simulink model "afe_inv_psm_with_hf_models"  (R2026a)
settings: Solver=ode23tb  StopTime=simlength  FixedStep=tc  MaxStep=glb_time.tc
values from neighbouring files (symbols this model uses):
  afe_ctrl = ctrl_afe_setup(glb_time.ts_afe, grid_emu.omega_grid_nom)    [init_model.m]
  afe_pwm_phase_shift_mod1 = 0    [init_model.m]
  CTRPIFF_CLIP_RELEASE = 0.001    [init_model.m]
  DThs_init = 0    [init_model.m]
  filters = setup_global_filters(glb_time.ts_afe, glb_time.ts_inv, glb_time.ts_dab, glb_time.tc)    [init_model.m]
  frt_data = frt_settings(test_index, test_subindex, asymmetric_error_type,      enable_frt_1, enable_frt_2, start_time_LVRT, deepPOSxi, deepPOSeta, deepNEGxi, deepNEGeta)    [init_model.m]
  glb_time = timing_setup(fpwm_afe, trgo_afe, fpwm_inv, trgo_inv, fpwm_single_phase_inv, trgo_single_phase_inv, fpwm_dab, trgo_dab,      fpwm_psfbc, trgo_psfbc, fpwm_isop_rail, trgo_isop_rail, fpwm_cllc, trgo_cllc, t_measure, tc_factor, tc_decimation, delay_pwm, dead_time_afe,      dead_time_inv, dead_time_single_phase_inv, dead_time_dab, dead_time_psfbc, dead_time_isop_rail, dead_time_cllc)    [init_model.m]
  grid_emu = grid_three_phase_emulator('Dyn11', delta_star, grid_nominal_power, application_voltage, us1, us2, fgrid,                  eq_grid_inductance, eq_grid_resistance, eta, ucc, i1m, p_iron, n1, n2, core_area, core_length, mur,                  up_xi_pu_ref, up_eta_pu_ref, un_xi_pu_ref, un_eta_pu_ref)    [init_model.m]
  i_react_pos_ref_2 = -ixi_ref_mod1*tan(acos(0.95))    [init_model.m]
  i_react_pos_ref_3 = ixi_ref_mod1*tan(acos(0.95))    [init_model.m]
  inv_pwm_phase_shift_mod1 = 0    [init_model.m]
  ixi_ref_mod1 = -0.85    [init_model.m]
  ki_align = 18    [init_model.m]
  kp_align = 0.25    [init_model.m]
  lim_down_align = -0.05    [init_model.m]
  lim_up_align = 0.05    [init_model.m]
  mavarage_filter_frequency_base_order = 2    [init_model.m]
  omega_m_sim = psm.omega_m_bez    [init_model.m]
  psm = psm_calculus_with_variants(application_voltage)    [init_model.m]
  psm_ctrl = ctrl_pmsm_setup(glb_time.ts_inv, psm.omega_bez, u_psm_scale, psm.Jm_norm)    [init_model.m]
  rms_tc = rms_filter_setup(rms_tc_obj)    [init_model.m]
  simlength = 1.75    [init_model.m]
  Tambient = 40    [init_model.m]
  time_aux_power_supply_fault = 1e3    (= 1000)    [init_model.m]
  time_gain_afe_module_1 = 1.0002    [init_model.m]
  time_gain_inv_module_2 = 1.001    [init_model.m]
  time_i_react_pos_ref_1 = start_time_LVRT + error_length + 0.335    [init_model.m]
  time_i_react_pos_ref_2 = time_i_react_pos_ref_1 + 0.5    (= 0.5)    [init_model.m]
  time_start_motor_control = 0.25    [init_model.m]
  torque_overload_factor = 1    [init_model.m]
  u_cm_comp_mod1 = 0    [init_model.m]
  u_psm_scale_ekf = sqrt(3)/2 * 2/3 * hwdata.inv.udc_nom/psm.ubez    [init_model.m]
undefined symbols (not defined in the file or in its folder): hf_power_cable_model, hwdata, magnitude, omega_m_bez, rpm_base, torque_base
libraries: fl_lib x136, nesl_utility x57, moving_average_filter x10, moving_average_filter_cc x8, ee_lib x5, sl_discontinuities x3, single_phase_transformer_lib x3, linear_double_integrator_observer_ccaller x2, discrete_time_low_pass_filter x2, threephase_inductor_lib x2, three_phase_pwm_modulator x2, three_phase_inverter_ideal_switch_based_model x2
(part 4 of 10)

== system afe_inv_psm_with_hf_models/grid/grid_emulator/threephase_vi_measures ==
  Bus Creator : BusCreator  Inputs=6
  Current Sensor : fl_lib/Electrical/Electrical Sensors/Current Sensor
  Current Sensor1 : fl_lib/Electrical/Electrical Sensors/Current Sensor
  Current Sensor2 : fl_lib/Electrical/Electrical Sensors/Current Sensor
  Electrical Reference1 : fl_lib/Electrical/Electrical Elements/Electrical Reference
  Voltage Sensor : fl_lib/Electrical/Electrical Sensors/Voltage Sensor
  Voltage Sensor1 : fl_lib/Electrical/Electrical Sensors/Voltage Sensor
  Voltage Sensor2 : fl_lib/Electrical/Electrical Sensors/Voltage Sensor
  i : Selector  InputPortWidth=6  IndexOptions=Index vector (dialog)  Indices=[4 5 6]  OutputSizes=1
  ia_grid : nesl_utility/PS-Simulink Converter  PhysicalDomain=network_engine_domain  SubClassName=ps_output  LeftPortType=input  RightPortType=output  PseudoPeriodic=off  Frequencies=[]  VectorFormat=1-D array  Unit=A  AffineConversion=off
  ib_grid : nesl_utility/PS-Simulink Converter  PhysicalDomain=network_engine_domain  SubClassName=ps_output  LeftPortType=input  RightPortType=output  PseudoPeriodic=off  Frequencies=[]  VectorFormat=1-D array  Unit=A  AffineConversion=off
  ic_grid : nesl_utility/PS-Simulink Converter  PhysicalDomain=network_engine_domain  SubClassName=ps_output  LeftPortType=input  RightPortType=output  PseudoPeriodic=off  Frequencies=[]  VectorFormat=1-D array  Unit=A  AffineConversion=off
  u : Selector  InputPortWidth=6  IndexOptions=Index vector (dialog)  Indices=[1 2 3]  OutputSizes=1
  ua_grid : nesl_utility/PS-Simulink Converter  PhysicalDomain=network_engine_domain  SubClassName=ps_output  LeftPortType=input  RightPortType=output  PseudoPeriodic=off  Frequencies=[]  VectorFormat=1-D array  Unit=V  AffineConversion=off
  ub_grid : nesl_utility/PS-Simulink Converter  PhysicalDomain=network_engine_domain  SubClassName=ps_output  LeftPortType=input  RightPortType=output  PseudoPeriodic=off  Frequencies=[]  VectorFormat=1-D array  Unit=V  AffineConversion=off
  uc_grid : nesl_utility/PS-Simulink Converter  PhysicalDomain=network_engine_domain  SubClassName=ps_output  LeftPortType=input  RightPortType=output  PseudoPeriodic=off  Frequencies=[]  VectorFormat=1-D array  Unit=V  AffineConversion=off
  Ua : PMIOPort  Side=Left
  ua : PMIOPort  Port=2  Side=Right
  Ub : PMIOPort  Port=3  Side=Left
  ub : PMIOPort  Port=4  Side=Right
  Uc : PMIOPort  Port=5  Side=Left
  uc : PMIOPort  Port=6  Side=Right
  tag scope: i_abc_line=global, u_abc_line=global
  wires:
  Bus Creator/1 -> i/1, u/1  "vi_data"
  ib_grid/1 -> Bus Creator/5  "ib"
  ia_grid/1 -> Bus Creator/4  "ia"
  ic_grid/1 -> Bus Creator/6  "ic"
  ua_grid/1 -> Bus Creator/1  "ua"
  ub_grid/1 -> Bus Creator/2  "ub"
  uc_grid/1 -> Bus Creator/3  "uc"
  i/1 -> [i_abc_line]
  u/1 -> [u_abc_line]
  connections:
  Current Sensor1/LConn1 -- Ub/RConn1 -- Voltage Sensor1/LConn1
  Electrical Reference1/LConn1 -- Voltage Sensor/RConn2 -- Voltage Sensor2/RConn2 -- Voltage Sensor1/RConn2
  Voltage Sensor/RConn1 -- ua_grid/LConn1
  Current Sensor/RConn2 -- ua/RConn1
  Voltage Sensor1/RConn1 -- ub_grid/LConn1
  Voltage Sensor2/LConn1 -- Current Sensor2/LConn1 -- Uc/RConn1
  Current Sensor/LConn1 -- Ua/RConn1 -- Voltage Sensor/LConn1
  Current Sensor1/RConn2 -- ub/RConn1
  Voltage Sensor2/RConn1 -- uc_grid/LConn1
  ib_grid/LConn1 -- Current Sensor1/RConn1
  ia_grid/LConn1 -- Current Sensor/RConn1
  ic_grid/LConn1 -- Current Sensor2/RConn1
  Current Sensor2/RConn2 -- uc/RConn1

== system afe_inv_psm_with_hf_models/power_cables_and_psm_high_frequency_models/power_cable_model_1/parasitic_lump_1 ==
  Cp1 : fl_lib/Electrical/Electrical Elements/Capacitor  c=hf_power_cable_model.Cp1 F  r=hf_power_cable_model.RCs1 Ohm  g=0 1/Ohm  i_specify=off  i_priority=None  i=0 A  i_nominal_specify=off  i_nominal_value=1  i_nominal_unit=A  v_specify=off  v_priority=None  v=0 V  v_nominal_specify=off  v_nominal_value=1  v_nominal_unit=V  vc_specify=off  vc_priority=High  vc=0 V  vc_nominal_specify=off  vc_nominal_value=1  vc_nominal_unit=V
  Cp2 : fl_lib/Electrical/Electrical Elements/Capacitor  Commented=on  c=hf_power_cable_model.Cp2 F  r=hf_power_cable_model.RCs2 Ohm  g=0 1/Ohm  i_specify=off  i_priority=None  i=0 A  i_nominal_specify=off  i_nominal_value=1  i_nominal_unit=A  v_specify=off  v_priority=None  v=0 V  v_nominal_specify=off  v_nominal_value=1  v_nominal_unit=V  vc_specify=off  vc_priority=High  vc=0 V  vc_nominal_specify=off  vc_nominal_value=1  vc_nominal_unit=V
  Electrical Reference : fl_lib/Electrical/Electrical Elements/Electrical Reference
  Ls1 : fl_lib/Electrical/Electrical Elements/Inductor  l=hf_power_cable_model.Ls1 H  r=hf_power_cable_model.Rs1 Ohm  g=1e-9 1/Ohm  i_specify=off  i_priority=None  i=0 A  i_nominal_specify=off  i_nominal_value=1  i_nominal_unit=A  v_specify=off  v_priority=None  v=0 V  v_nominal_specify=off  v_nominal_value=1  v_nominal_unit=V  i_L_specify=off  i_L_priority=High  i_L=0 A  i_L_nominal_specify=off  i_L_nominal_value=1  i_L_nominal_unit=A
  Rp1 : fl_lib/Electrical/Electrical Elements/Resistor  Commented=on  R=hf_power_cable_model.Rp1 Ohm  i_specify=off  i_priority=None  i=0 A  i_nominal_specify=off  i_nominal_value=1  i_nominal_unit=A  v_specify=off  v_priority=None  v=0 V  v_nominal_specify=off  v_nominal_value=1  v_nominal_unit=V
  u1 : PMIOPort  Side=Left
  u2 : PMIOPort  Port=2  Side=Right
  connections:
  Ls1/LConn1 -- Cp2/LConn1 -- u1/RConn1
  Rp1/RConn1 -- Cp2/RConn1 -- Electrical Reference/LConn1 -- Cp1/RConn1
  u2/RConn1 -- Rp1/LConn1 -- Ls1/RConn1 -- Cp1/LConn1

== system afe_inv_psm_with_hf_models/power_cables_and_psm_high_frequency_models/power_cable_model_1/parasitic_lump_2 ==
  Cp1 : fl_lib/Electrical/Electrical Elements/Capacitor  c=hf_power_cable_model.Cp1 F  r=hf_power_cable_model.RCs1 Ohm  g=0 1/Ohm  i_specify=off  i_priority=None  i=0 A  i_nominal_specify=off  i_nominal_value=1  i_nominal_unit=A  v_specify=off  v_priority=None  v=0 V  v_nominal_specify=off  v_nominal_value=1  v_nominal_unit=V  vc_specify=off  vc_priority=High  vc=0 V  vc_nominal_specify=off  vc_nominal_value=1  vc_nominal_unit=V
  Cp2 : fl_lib/Electrical/Electrical Elements/Capacitor  Commented=on  c=hf_power_cable_model.Cp2 F  r=hf_power_cable_model.RCs2 Ohm  g=0 1/Ohm  i_specify=off  i_priority=None  i=0 A  i_nominal_specify=off  i_nominal_value=1  i_nominal_unit=A  v_specify=off  v_priority=None  v=0 V  v_nominal_specify=off  v_nominal_value=1  v_nominal_unit=V  vc_specify=off  vc_priority=High  vc=0 V  vc_nominal_specify=off  vc_nominal_value=1  vc_nominal_unit=V
  Electrical Reference : fl_lib/Electrical/Electrical Elements/Electrical Reference
  Ls1 : fl_lib/Electrical/Electrical Elements/Inductor  l=hf_power_cable_model.Ls1 H  r=hf_power_cable_model.Rs1 Ohm  g=1e-9 1/Ohm  i_specify=off  i_priority=None  i=0 A  i_nominal_specify=off  i_nominal_value=1  i_nominal_unit=A  v_specify=off  v_priority=None  v=0 V  v_nominal_specify=off  v_nominal_value=1  v_nominal_unit=V  i_L_specify=off  i_L_priority=High  i_L=0 A  i_L_nominal_specify=off  i_L_nominal_value=1  i_L_nominal_unit=A
  Rp1 : fl_lib/Electrical/Electrical Elements/Resistor  Commented=on  R=hf_power_cable_model.Rp1 Ohm  i_specify=off  i_priority=None  i=0 A  i_nominal_specify=off  i_nominal_value=1  i_nominal_unit=A  v_specify=off  v_priority=None  v=0 V  v_nominal_specify=off  v_nominal_value=1  v_nominal_unit=V
  u1 : PMIOPort  Side=Left
  u2 : PMIOPort  Port=2  Side=Right
  connections:
  Cp1/LConn1 -- Ls1/RConn1 -- Rp1/LConn1 -- u2/RConn1
  Cp1/RConn1 -- Electrical Reference/LConn1 -- Cp2/RConn1 -- Rp1/RConn1
  u1/RConn1 -- Cp2/LConn1 -- Ls1/LConn1

== system afe_inv_psm_with_hf_models/power_cables_and_psm_high_frequency_models/power_cable_model_2/parasitic_lump_1 ==
  Cp1 : fl_lib/Electrical/Electrical Elements/Capacitor  c=hf_power_cable_model.Cp1 F  r=hf_power_cable_model.RCs1 Ohm  g=0 1/Ohm  i_specify=off  i_priority=None  i=0 A  i_nominal_specify=off  i_nominal_value=1  i_nominal_unit=A  v_specify=off  v_priority=None  v=0 V  v_nominal_specify=off  v_nominal_value=1  v_nominal_unit=V  vc_specify=off  vc_priority=High  vc=0 V  vc_nominal_specify=off  vc_nominal_value=1  vc_nominal_unit=V
  Cp2 : fl_lib/Electrical/Electrical Elements/Capacitor  Commented=on  c=hf_power_cable_model.Cp2 F  r=hf_power_cable_model.RCs2 Ohm  g=0 1/Ohm  i_specify=off  i_priority=None  i=0 A  i_nominal_specify=off  i_nominal_value=1  i_nominal_unit=A  v_specify=off  v_priority=None  v=0 V  v_nominal_specify=off  v_nominal_value=1  v_nominal_unit=V  vc_specify=off  vc_priority=High  vc=0 V  vc_nominal_specify=off  vc_nominal_value=1  vc_nominal_unit=V
  Electrical Reference : fl_lib/Electrical/Electrical Elements/Electrical Reference
  Ls1 : fl_lib/Electrical/Electrical Elements/Inductor  l=hf_power_cable_model.Ls1 H  r=hf_power_cable_model.Rs1 Ohm  g=1e-9 1/Ohm  i_specify=off  i_priority=None  i=0 A  i_nominal_specify=off  i_nominal_value=1  i_nominal_unit=A  v_specify=off  v_priority=None  v=0 V  v_nominal_specify=off  v_nominal_value=1  v_nominal_unit=V  i_L_specify=off  i_L_priority=High  i_L=0 A  i_L_nominal_specify=off  i_L_nominal_value=1  i_L_nominal_unit=A
  Rp1 : fl_lib/Electrical/Electrical Elements/Resistor  Commented=on  R=hf_power_cable_model.Rp1 Ohm  i_specify=off  i_priority=None  i=0 A  i_nominal_specify=off  i_nominal_value=1  i_nominal_unit=A  v_specify=off  v_priority=None  v=0 V  v_nominal_specify=off  v_nominal_value=1  v_nominal_unit=V
  u1 : PMIOPort  Side=Left
  u2 : PMIOPort  Port=2  Side=Right
  connections:
  Cp1/LConn1 -- Ls1/RConn1 -- Rp1/LConn1 -- u2/RConn1
  Cp1/RConn1 -- Electrical Reference/LConn1 -- Cp2/RConn1 -- Rp1/RConn1
  u1/RConn1 -- Cp2/LConn1 -- Ls1/LConn1

== system afe_inv_psm_with_hf_models/power_cables_and_psm_high_frequency_models/power_cable_model_2/parasitic_lump_2 ==
  Cp1 : fl_lib/Electrical/Electrical Elements/Capacitor  c=hf_power_cable_model.Cp1 F  r=hf_power_cable_model.RCs1 Ohm  g=0 1/Ohm  i_specify=off  i_priority=None  i=0 A  i_nominal_specify=off  i_nominal_value=1  i_nominal_unit=A  v_specify=off  v_priority=None  v=0 V  v_nominal_specify=off  v_nominal_value=1  v_nominal_unit=V  vc_specify=off  vc_priority=High  vc=0 V  vc_nominal_specify=off  vc_nominal_value=1  vc_nominal_unit=V
  Cp2 : fl_lib/Electrical/Electrical Elements/Capacitor  Commented=on  c=hf_power_cable_model.Cp2 F  r=hf_power_cable_model.RCs2 Ohm  g=0 1/Ohm  i_specify=off  i_priority=None  i=0 A  i_nominal_specify=off  i_nominal_value=1  i_nominal_unit=A  v_specify=off  v_priority=None  v=0 V  v_nominal_specify=off  v_nominal_value=1  v_nominal_unit=V  vc_specify=off  vc_priority=High  vc=0 V  vc_nominal_specify=off  vc_nominal_value=1  vc_nominal_unit=V
  Electrical Reference : fl_lib/Electrical/Electrical Elements/Electrical Reference
  Ls1 : fl_lib/Electrical/Electrical Elements/Inductor  l=hf_power_cable_model.Ls1 H  r=hf_power_cable_model.Rs1 Ohm  g=1e-9 1/Ohm  i_specify=off  i_priority=None  i=0 A  i_nominal_specify=off  i_nominal_value=1  i_nominal_unit=A  v_specify=off  v_priority=None  v=0 V  v_nominal_specify=off  v_nominal_value=1  v_nominal_unit=V  i_L_specify=off  i_L_priority=High  i_L=0 A  i_L_nominal_specify=off  i_L_nominal_value=1  i_L_nominal_unit=A
  Rp1 : fl_lib/Electrical/Electrical Elements/Resistor  Commented=on  R=hf_power_cable_model.Rp1 Ohm  i_specify=off  i_priority=None  i=0 A  i_nominal_specify=off  i_nominal_value=1  i_nominal_unit=A  v_specify=off  v_priority=None  v=0 V  v_nominal_specify=off  v_nominal_value=1  v_nominal_unit=V
  u1 : PMIOPort  Side=Left
  u2 : PMIOPort  Port=2  Side=Right
  connections:
  Ls1/LConn1 -- Cp2/LConn1 -- u1/RConn1
  Cp2/RConn1 -- Electrical Reference/LConn1 -- Rp1/RConn1 -- Cp1/RConn1
  u2/RConn1 -- Rp1/LConn1 -- Ls1/RConn1 -- Cp1/LConn1

== system afe_inv_psm_with_hf_models/power_cables_and_psm_high_frequency_models/power_cable_model_3/parasitic_lump_1 ==
  Cp1 : fl_lib/Electrical/Electrical Elements/Capacitor  c=hf_power_cable_model.Cp1 F  r=hf_power_cable_model.RCs1 Ohm  g=0 1/Ohm  i_specify=off  i_priority=None  i=0 A  i_nominal_specify=off  i_nominal_value=1  i_nominal_unit=A  v_specify=off  v_priority=None  v=0 V  v_nominal_specify=off  v_nominal_value=1  v_nominal_unit=V  vc_specify=off  vc_priority=High  vc=0 V  vc_nominal_specify=off  vc_nominal_value=1  vc_nominal_unit=V
  Cp2 : fl_lib/Electrical/Electrical Elements/Capacitor  Commented=on  c=hf_power_cable_model.Cp2 F  r=hf_power_cable_model.RCs2 Ohm  g=0 1/Ohm  i_specify=off  i_priority=None  i=0 A  i_nominal_specify=off  i_nominal_value=1  i_nominal_unit=A  v_specify=off  v_priority=None  v=0 V  v_nominal_specify=off  v_nominal_value=1  v_nominal_unit=V  vc_specify=off  vc_priority=High  vc=0 V  vc_nominal_specify=off  vc_nominal_value=1  vc_nominal_unit=V
  Electrical Reference : fl_lib/Electrical/Electrical Elements/Electrical Reference
  Ls1 : fl_lib/Electrical/Electrical Elements/Inductor  l=hf_power_cable_model.Ls1 H  r=hf_power_cable_model.Rs1 Ohm  g=1e-9 1/Ohm  i_specify=off  i_priority=None  i=0 A  i_nominal_specify=off  i_nominal_value=1  i_nominal_unit=A  v_specify=off  v_priority=None  v=0 V  v_nominal_specify=off  v_nominal_value=1  v_nominal_unit=V  i_L_specify=off  i_L_priority=High  i_L=0 A  i_L_nominal_specify=off  i_L_nominal_value=1  i_L_nominal_unit=A
  Rp1 : fl_lib/Electrical/Electrical Elements/Resistor  Commented=on  R=hf_power_cable_model.Rp1 Ohm  i_specify=off  i_priority=None  i=0 A  i_nominal_specify=off  i_nominal_value=1  i_nominal_unit=A  v_specify=off  v_priority=None  v=0 V  v_nominal_specify=off  v_nominal_value=1  v_nominal_unit=V
  u1 : PMIOPort  Side=Left
  u2 : PMIOPort  Port=2  Side=Right
  connections:
  Ls1/LConn1 -- Cp2/LConn1 -- u1/RConn1
  Cp2/RConn1 -- Electrical Reference/LConn1 -- Rp1/RConn1 -- Cp1/RConn1
  u2/RConn1 -- Rp1/LConn1 -- Ls1/RConn1 -- Cp1/LConn1

== system afe_inv_psm_with_hf_models/power_cables_and_psm_high_frequency_models/power_cable_model_3/parasitic_lump_2 ==
  Cp1 : fl_lib/Electrical/Electrical Elements/Capacitor  c=hf_power_cable_model.Cp1 F  r=hf_power_cable_model.RCs1 Ohm  g=0 1/Ohm  i_specify=off  i_priority=None  i=0 A  i_nominal_specify=off  i_nominal_value=1  i_nominal_unit=A  v_specify=off  v_priority=None  v=0 V  v_nominal_specify=off  v_nominal_value=1  v_nominal_unit=V  vc_specify=off  vc_priority=High  vc=0 V  vc_nominal_specify=off  vc_nominal_value=1  vc_nominal_unit=V
  Cp2 : fl_lib/Electrical/Electrical Elements/Capacitor  Commented=on  c=hf_power_cable_model.Cp2 F  r=hf_power_cable_model.RCs2 Ohm  g=0 1/Ohm  i_specify=off  i_priority=None  i=0 A  i_nominal_specify=off  i_nominal_value=1  i_nominal_unit=A  v_specify=off  v_priority=None  v=0 V  v_nominal_specify=off  v_nominal_value=1  v_nominal_unit=V  vc_specify=off  vc_priority=High  vc=0 V  vc_nominal_specify=off  vc_nominal_value=1  vc_nominal_unit=V
  Electrical Reference : fl_lib/Electrical/Electrical Elements/Electrical Reference
  Ls1 : fl_lib/Electrical/Electrical Elements/Inductor  l=hf_power_cable_model.Ls1 H  r=hf_power_cable_model.Rs1 Ohm  g=1e-9 1/Ohm  i_specify=off  i_priority=None  i=0 A  i_nominal_specify=off  i_nominal_value=1  i_nominal_unit=A  v_specify=off  v_priority=None  v=0 V  v_nominal_specify=off  v_nominal_value=1  v_nominal_unit=V  i_L_specify=off  i_L_priority=High  i_L=0 A  i_L_nominal_specify=off  i_L_nominal_value=1  i_L_nominal_unit=A
  Rp1 : fl_lib/Electrical/Electrical Elements/Resistor  Commented=on  R=hf_power_cable_model.Rp1 Ohm  i_specify=off  i_priority=None  i=0 A  i_nominal_specify=off  i_nominal_value=1  i_nominal_unit=A  v_specify=off  v_priority=None  v=0 V  v_nominal_specify=off  v_nominal_value=1  v_nominal_unit=V
  u1 : PMIOPort  Side=Left
  u2 : PMIOPort  Port=2  Side=Right
  connections:
  Cp1/LConn1 -- Ls1/RConn1 -- Rp1/LConn1 -- u2/RConn1
  Cp1/RConn1 -- Rp1/RConn1 -- Electrical Reference/LConn1 -- Cp2/RConn1
  u1/RConn1 -- Cp2/LConn1 -- Ls1/LConn1

== system afe_inv_psm_with_hf_models/scopes/cable_effects/rms ==
  in : Inport
  Gain : Gain  Gain=rms_tc.n1-1
  Gain1 : Gain  Gain=1/rms_tc.n1
  Math Function : Math  Operator=magnitude^2  SignedPower=on
  Sqrt : Sqrt
  Sum : Sum  Inputs=|++
  Unit Delay : UnitDelay  SampleTime=glb_time.tc
  out : Outport  VectorParamsAs1DForOutWhenUnconnected=off
  wires:
  in/1 -> Math Function/1
  Sum/1 -> Gain1/1
  Gain1/1 -> Sqrt/1, Unit Delay/1
  Unit Delay/1 -> Gain/1
  Math Function/1 -> Sum/1
  Sqrt/1 -> out/1
  Gain/1 -> Sum/2

== system afe_inv_psm_with_hf_models/afe_abc_inv_psm_mod1/AFE_control/afe_control/FRT-VDE4110 ==
  Constant : Constant  Value=0
  FRT-Detection : Subsystem
  FRT-PosNegReactiveCurrentReferences : Subsystem
  Terminator : Terminator
  Terminator1 : Terminator
  frt_detection_output : Scope  NumInputPorts=3
      settings: ActiveDisplayYMinimum=-0.12499999999999997  ActiveDisplayYMaximum=1.125
  tag scope: frt_active=scoped, pwr_lim_enable=scoped
  wires:
  [v_grid_pos_xi_avg] -> FRT-PosNegReactiveCurrentReferences/1(In1)
  [v_grid_neg_xi_avg] -> FRT-PosNegReactiveCurrentReferences/3(In3)
  [v_grid_neg_eta_avg] -> FRT-PosNegReactiveCurrentReferences/4(In4)
  [v_grid_pos_eta_avg] -> FRT-PosNegReactiveCurrentReferences/2(In2)
  FRT-Detection/4(frt_active) -> frt_detection_output/2, [frt_active]  "frt_active"
  FRT-Detection/5(pwr_lim_enable) -> frt_detection_output/3, [pwr_lim_enable]  "pwr_lim_enable"
  FRT-Detection/2(frt_state) -> frt_detection_output/1  "frt_state"
  Constant/1 -> FRT-Detection/1(red_dyn_enabled)
  FRT-Detection/1(frt_exceeded) -> Terminator/1
  FRT-Detection/3(red_dyn_active) -> Terminator1/1

== system afe_inv_psm_with_hf_models/afe_abc_inv_psm_mod1/AFE_control/afe_control/current_ctrl ==
  i_xi_ref : Inport
  Demux : Demux  Outputs=3
  current_transformation : Subsystem
  inner_current_ctrl : Subsystem
  xieta2abc : Subsystem
  uabg_out : Outport
  wires:
  Demux/1 -> current_transformation/1(is_a_pu)  "is_a"
  Demux/2 -> current_transformation/2(is_b_pu)  "is_b"
  Demux/3 -> current_transformation/3(is_c_pu)  "is_c"
  [isd_abc_pu] -> Demux/1
  [phase_grid_pll] -> xieta2abc/5(phase)
  xieta2abc/1(i_abc) -> inner_current_ctrl/1(In1)
  [isd_abc_pu] -> inner_current_ctrl/2(is_abc)
  inner_current_ctrl/1(uabg) -> uabg_out/1
  i_xi_ref/1 -> xieta2abc/1(pos_xi)  "i_xi_ref"
  [i_stack_neg_eta_ref] -> xieta2abc/4(neg_eta)
  [i_stack_neg_xi_ref] -> xieta2abc/3(neg_xi)
  [i_stack_pos_eta_ref] -> xieta2abc/2(pos_eta)

== system afe_inv_psm_with_hf_models/afe_abc_inv_psm_mod1/AFE_control/afe_control/data_to_worspace_module_1 ==
  Bus Creator : BusCreator  Inputs=5
  dq_pll : Subsystem
  inner_current_tracking : Subsystem
  pwr_meter : Subsystem
  sequences_data : Subsystem
  m : Outport
  wires:
  Bus Creator/1 -> m/1
  sequences_data/1(m_seq) -> Bus Creator/1  "sequences_data"
  pwr_meter/1(m_pwr_meter) -> Bus Creator/2  "pwr_meter"
  inner_current_tracking/1(m_inner_current_tracking) -> Bus Creator/3  "m_inner_current_tracking"
  [local_time] -> Bus Creator/5  "local_time"
  dq_pll/1(dqPLLs) -> Bus Creator/4  "dq_pll"

== system afe_inv_psm_with_hf_models/afe_abc_inv_psm_mod1/AFE_control/afe_control/grid_current_sequences_and_reactive_pwr_ctrl ==
  ig_abc_pu : Inport
  current_sequence_avg : Subsystem
  grid_current_sampling_and_alpha_beta_transformation : Subsystem
  i_alphabeta2xieta : Subsystem
  sequences_current_control : Subsystem
  tag scope: i_grid_neg_eta_avg=scoped, i_grid_neg_xi_avg=scoped, i_grid_pos_eta_avg=scoped, i_grid_pos_xi_avg=scoped
  wires:
  i_alphabeta2xieta/1(xi) -> current_sequence_avg/1(i_grid_pos_xi)
  i_alphabeta2xieta/3(v_grid_neg_xi) -> current_sequence_avg/3(i_grid_neg_xi)
  i_alphabeta2xieta/4(e) -> current_sequence_avg/4(i_grid_neg_eta)
  current_sequence_avg/4(i_grid_neg_eta_avg) -> sequences_current_control/4(i_neg_eta), [i_grid_neg_eta_avg]
  ig_abc_pu/1 -> grid_current_sampling_and_alpha_beta_transformation/1(ig_abc)
  i_alphabeta2xieta/2(v_grid_pos_eta) -> current_sequence_avg/2(i_grid_pos_eta)
  current_sequence_avg/1(i_grid_pos_xi_avg) -> [i_grid_pos_xi_avg], sequences_current_control/1(i_pos_xi)
  current_sequence_avg/2(i_grid_pos_eta_avg) -> [i_grid_pos_eta_avg], sequences_current_control/2(i_pos_eta)
  [phase_grid_pll] -> i_alphabeta2xieta/3(gamma)
  grid_current_sampling_and_alpha_beta_transformation/2(i_grid_beta) -> i_alphabeta2xieta/2(beta)
  grid_current_sampling_and_alpha_beta_transformation/1(i_grid_alpha) -> i_alphabeta2xieta/1(alpha)
  current_sequence_avg/3(i_grid_neg_xi_avg) -> sequences_current_control/3(i_neg_xi), [i_grid_neg_xi_avg]

== system afe_inv_psm_with_hf_models/afe_abc_inv_psm_mod1/AFE_control/afe_control/grid_phase_acquisition ==
  grid_phase : Inport
  Quantizer : Quantizer  QuantizationInterval=adc_quantization
  Unit Delay : UnitDelay  SampleTime=-1
  Zero-Order Hold : ZeroOrderHold  SampleTime=-1
  grid_phased : Outport
  wires:
  Zero-Order Hold/1 -> Quantizer/1
  Unit Delay/1 -> grid_phased/1
  grid_phase/1 -> Zero-Order Hold/1
  Quantizer/1 -> Unit Delay/1

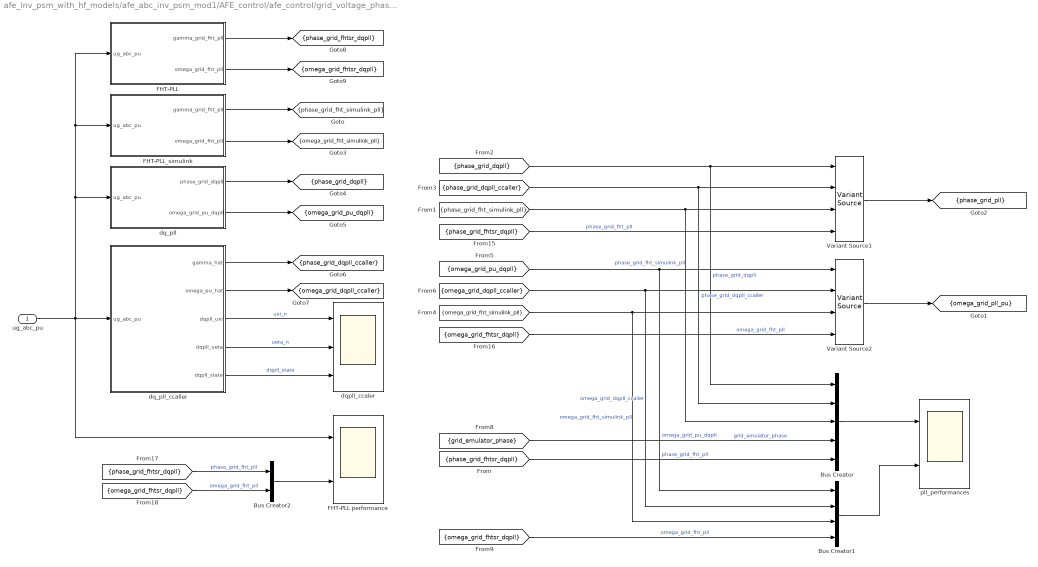
== system afe_inv_psm_with_hf_models/afe_abc_inv_psm_mod1/AFE_control/afe_control/grid_voltage_phase_lock_loops ==
  ug_abc_pu : Inport
  Bus Creator : BusCreator  Inputs=5
  Bus Creator1 : BusCreator  Inputs=4
  Bus Creator2 : BusCreator  Inputs=2
  FHT-PLL : Subsystem
  FHT-PLL performance : Scope  NumInputPorts=2
      settings: ActiveDisplayYMinimum=-1.251220703125  ActiveDisplayYMaximum=1.251220703125  DataLoggingVariableName=ScopeData8
  FHT-PLL_simulink : Subsystem
  Variant Source1 : VariantSource  VariantControls={use_dq_pll_mode1 == 1, use_dq_pll_mode2 == 1, use_dq_pll_mode3 == 1, use_dq_pll_mode4 == 1}
  Variant Source2 : VariantSource  VariantControls={use_dq_pll_mode1 == 1, use_dq_pll_mode2 == 1, use_dq_pll_mode3 == 1, use_dq_pll_mode4 == 1}
  dq_pll : Subsystem
  dq_pll_ccaller : Subsystem
  dqpll_ccaler : Scope  NumInputPorts=3
      settings: ActiveDisplayYMinimum=-0.88802937790751446  ActiveDisplayYMaximum=4.5431143753230572  DataLoggingVariableName=ScopeData4
  pll_performances : Scope  NumInputPorts=2
      settings: ActiveDisplayYMinimum=-3.9264641704366507  ActiveDisplayYMaximum=3.9264746341683896  DataLoggingVariableName=ScopeData34
  tag scope: omega_grid_dqpll_ccaller=scoped, omega_grid_fht_simulink_pll=scoped, omega_grid_fhtsr_dqpll=scoped, omega_grid_pll_pu=scoped, omega_grid_pu_dqpll=scoped, phase_grid_dqpll=scoped, phase_grid_dqpll_ccaller=scoped, phase_grid_fht_simulink_pll=scoped, phase_grid_fhtsr_dqpll=scoped, phase_grid_pll=scoped
  wires:
  Variant Source1/1 -> [phase_grid_pll]
  FHT-PLL_simulink/1(gamma_grid_fht_pll) -> [phase_grid_fht_simulink_pll]
  FHT-PLL_simulink/2(omega_grid_fht_pll) -> [omega_grid_fht_simulink_pll]
  dq_pll/2(omega_grid_pu_dqpll) -> [omega_grid_pu_dqpll]
  dq_pll/1(phase_grid_dqpll) -> [phase_grid_dqpll]
  dq_pll_ccaller/1(gamma_hat) -> [phase_grid_dqpll_ccaller]
  dq_pll_ccaller/2(omega_pu_hat) -> [omega_grid_dqpll_ccaller]
  [phase_grid_dqpll] -> Variant Source1/1, Bus Creator/1  "phase_grid_dqpll"
  [phase_grid_dqpll_ccaller] -> Bus Creator/2, Variant Source1/2  "phase_grid_dqpll_ccaller"
  [phase_grid_fht_simulink_pll] -> Bus Creator/3, Variant Source1/3  "phase_grid_fht_simulink_pll"
  [omega_grid_pu_dqpll] -> Variant Source2/1, Bus Creator1/1  "omega_grid_pu_dqpll"
  [omega_grid_dqpll_ccaller] -> Variant Source2/2, Bus Creator1/2  "omega_grid_dqpll_ccaller"
  [omega_grid_fht_simulink_pll] -> Variant Source2/3, Bus Creator1/3  "omega_grid_fht_simulink_pll"
  Variant Source2/1 -> [omega_grid_pll_pu]
  dq_pll_ccaller/3(dqpll_uxi) -> dqpll_ccaler/1  "uxi_n"
  dq_pll_ccaller/4(dqpll_ueta) -> dqpll_ccaler/2  "ueta_n"
  dq_pll_ccaller/5(dqpll_state) -> dqpll_ccaler/3  "dqpll_state"
  ug_abc_pu/1 -> FHT-PLL performance/1, dq_pll/1(ug_abc_pu), FHT-PLL_simulink/1(ug_abc_pu), FHT-PLL/1(ug_abc_pu), dq_pll_ccaller/1(ug_abc_pu)
  Bus Creator/1 -> pll_performances/1
  Bus Creator1/1 -> pll_performances/2
  [grid_emulator_phase] -> Bus Creator/4  "grid_emulator_phase"
  FHT-PLL/2(omega_grid_fht_pll) -> [omega_grid_fhtsr_dqpll]
  FHT-PLL/1(gamma_grid_fht_pll) -> [phase_grid_fhtsr_dqpll]
  [phase_grid_fhtsr_dqpll] -> Bus Creator/5  "phase_grid_fht_pll"
  [omega_grid_fhtsr_dqpll] -> Bus Creator1/4  "omega_grid_fht_pll"
  [phase_grid_fhtsr_dqpll] -> Variant Source1/4  "phase_grid_fht_pll"
  [omega_grid_fhtsr_dqpll] -> Variant Source2/4  "omega_grid_fht_pll"
  Bus Creator2/1 -> FHT-PLL performance/2
  [omega_grid_fhtsr_dqpll] -> Bus Creator2/2  "omega_grid_fht_pll"
  [phase_grid_fhtsr_dqpll] -> Bus Creator2/1  "phase_grid_fht_pll"

== system afe_inv_psm_with_hf_models/afe_abc_inv_psm_mod1/AFE_control/afe_control/grid_voltage_sequences ==
  grid_voltage_sampling_and_alpha_beta_transformation : Subsystem
  v_alphabeta2xieta : Subsystem
  voltage_sequence_avg : Subsystem
  tag scope: ug_alpha_pu=scoped, ug_beta_pu=scoped, v_grid_neg_eta_avg=scoped, v_grid_neg_xi_avg=scoped, v_grid_pos_eta_avg=scoped, v_grid_pos_xi_avg=scoped
  wires:
  v_alphabeta2xieta/4(v_grid_neg_eta) -> voltage_sequence_avg/4(v_grid_neg_eta)  "neg_eta"
  v_alphabeta2xieta/2(eta) -> voltage_sequence_avg/2(v_grid_pos_eta)  "pos_eta"
  [phase_grid_pll] -> v_alphabeta2xieta/3(gamma)
  v_alphabeta2xieta/3(v_grid_neg_xi) -> voltage_sequence_avg/3(v_grid_neg_xi)  "neg_xi"
  voltage_sequence_avg/3(v_grid_neg_xi_avg) -> [v_grid_neg_xi_avg]
  voltage_sequence_avg/2(v_grid_pos_eta_avg) -> [v_grid_pos_eta_avg]
  voltage_sequence_avg/4(v_grid_neg_eta_avg) -> [v_grid_neg_eta_avg]
  grid_voltage_sampling_and_alpha_beta_transformation/2(u_grid_beta) -> [ug_beta_pu], v_alphabeta2xieta/2(beta)
  voltage_sequence_avg/1(v_grid_pos_xi_avg) -> [v_grid_pos_xi_avg]
  v_alphabeta2xieta/1(xi) -> voltage_sequence_avg/1(v_grid_pos_xi)  "pos_xi"
  grid_voltage_sampling_and_alpha_beta_transformation/1(u_grid_alpha) -> [ug_alpha_pu], v_alphabeta2xieta/1(alpha)
  [ugd_abc_pu] -> grid_voltage_sampling_and_alpha_beta_transformation/1(v_abc)

== system afe_inv_psm_with_hf_models/afe_abc_inv_psm_mod1/AFE_control/afe_control/i_xi_ref ==
  Constant1 : Constant  Value=ixi_ref_mod1
  Constant2 : Constant  Value=0
  Delay : Delay  DelayLength=floor(0.25/glb_time.ts_afe)
  Switch : Switch  Criteria=u2 > Threshold  SaturateOnIntegerOverflow=off  InputSameDT=off
  Switch1 : Switch  Criteria=u2 > Threshold  SaturateOnIntegerOverflow=off  InputSameDT=off
  Variant Source : VariantSource  VariantControls={false, true}
  discrete-time-low-pass-filter : discrete_time_low_pass_filter/discrete-time-low-pass-filter  tau=0.125  ts=glb_time.ts_afe
  i_xi_ref : Outport
  wires:
  Constant1/1 -> Switch/3  "i_xi_ref"
  Constant2/1 -> Switch/1
  [pwr_lim_enable] -> Switch/2
  [pwr_lim_enable] -> Delay/1
  Switch/1 -> discrete-time-low-pass-filter/1, Variant Source/2, Switch1/3
  Delay/1 -> Switch1/2
  discrete-time-low-pass-filter/1 -> Switch1/1
  Switch1/1 -> Variant Source/1
  Variant Source/1 -> i_xi_ref/1

== system afe_inv_psm_with_hf_models/afe_abc_inv_psm_mod1/AFE_control/afe_control/ig afe quantizzation and one step delay ==
  ig_abc_pu : Inport
  Demux1 : Demux  Outputs=3
  Mux1 : Mux  Inputs=3
  ig afe quantizzation and one step delay : Subsystem
  igd_abc_pu : Outport
  wires:
  Demux1/1 -> ig afe quantizzation and one step delay/1(ig_u_pu)
  Demux1/2 -> ig afe quantizzation and one step delay/2(ig_v_pu)
  ig_abc_pu/1 -> Demux1/1
  Mux1/1 -> igd_abc_pu/1
  Demux1/3 -> ig afe quantizzation and one step delay/3(ig_w_pu)
  ig afe quantizzation and one step delay/2(igd_v_pu) -> Mux1/2
  ig afe quantizzation and one step delay/1(igd_u_pu) -> Mux1/1
  ig afe quantizzation and one step delay/3(igd_w_pu) -> Mux1/3

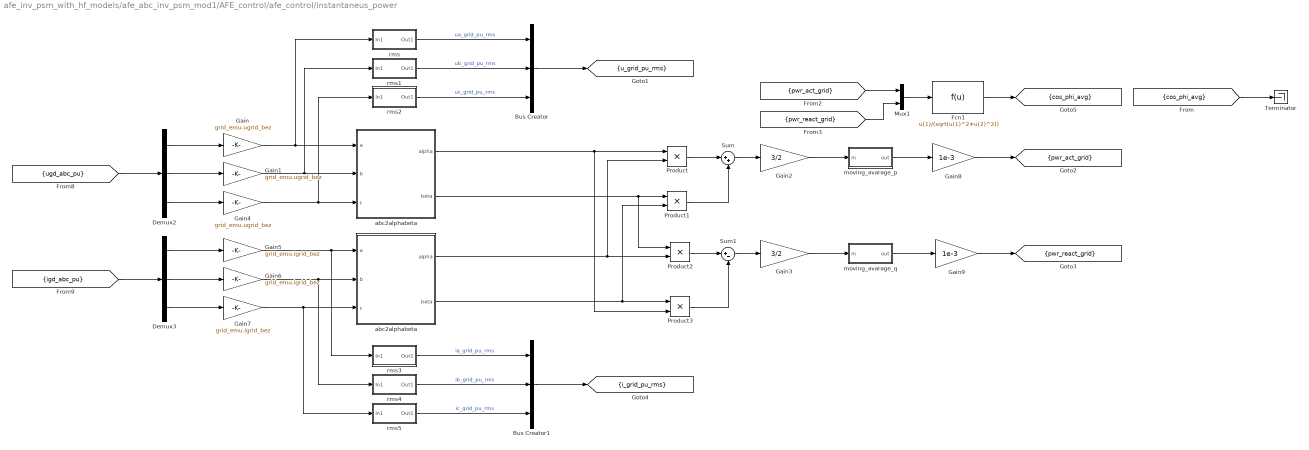
== system afe_inv_psm_with_hf_models/afe_abc_inv_psm_mod1/AFE_control/afe_control/instantaneus_power ==
  Bus Creator : BusCreator  Inputs=3
  Bus Creator1 : BusCreator  Inputs=3
  Demux2 : Demux  Outputs=3
  Demux3 : Demux  Outputs=3
  Fcn1 : Fcn  Expr=u(1)/(sqrt(u(1)^2+u(2)^2))
  Gain : Gain  Gain=grid_emu.ugrid_bez
  Gain1 : Gain  Gain=grid_emu.ugrid_bez
  Gain2 : Gain  Gain=3/2
  Gain3 : Gain  Gain=3/2
  Gain4 : Gain  Gain=grid_emu.ugrid_bez
  Gain5 : Gain  Gain=grid_emu.igrid_bez
  Gain6 : Gain  Gain=grid_emu.igrid_bez
  Gain7 : Gain  Gain=grid_emu.igrid_bez
  Gain8 : Gain  Gain=1e-3
  Gain9 : Gain  Gain=1e-3
  Mux1 : Mux  Inputs=2
  Product{,1..3} (4 alike) : Product  RndMeth=Zero
  Sum : Sum  Inputs=|++
  Sum1 : Sum  Inputs=|+-
  Terminator : Terminator
  abc2alphabeta : Subsystem
  "abc2alphabeta " : Subsystem
  moving_avarage_p : Subsystem
  moving_avarage_q : Subsystem
  rms : Subsystem
  rms1 : Subsystem
  rms2 : Subsystem
  rms3 : Subsystem
  rms4 : Subsystem
  rms5 : Subsystem
  tag scope: cos_phi_avg=scoped, i_grid_pu_rms=scoped, pwr_act_grid=scoped, pwr_react_grid=scoped, u_grid_pu_rms=scoped
  wires:
  abc2alphabeta/2("beta ") -> Product1/1, Product2/1
  "abc2alphabeta "/2("beta ") -> Product1/2, Product3/1
  abc2alphabeta/1("alpha ") -> Product3/2, Product/1
  "abc2alphabeta "/1("alpha ") -> Product2/2, Product/2
  Product/1 -> Sum/1
  Product1/1 -> Sum/2
  Product2/1 -> Sum1/1
  Product3/1 -> Sum1/2
  Sum1/1 -> Gain3/1
  Sum/1 -> Gain2/1
  Gain2/1 -> moving_avarage_p/1(in)
  Gain3/1 -> moving_avarage_q/1(in)
  [pwr_react_grid] -> Mux1/2
  Mux1/1 -> Fcn1/1
  Fcn1/1 -> [cos_phi_avg]
  [pwr_act_grid] -> Mux1/1
  rms/1(Out1) -> Bus Creator/1  "ua_grid_pu_rms"
  rms2/1(Out1) -> Bus Creator/3  "uc_grid_pu_rms"
  rms1/1(Out1) -> Bus Creator/2  "ub_grid_pu_rms"
  moving_avarage_p/1(out) -> Gain8/1
  moving_avarage_q/1(out) -> Gain9/1
  Demux2/1 -> Gain/1
  Demux2/2 -> Gain1/1
  Demux2/3 -> Gain4/1
  Demux3/1 -> Gain5/1
  Demux3/2 -> Gain6/1
  Demux3/3 -> Gain7/1
  Gain/1 -> rms/1(In1), abc2alphabeta/1(a)
  Gain1/1 -> rms1/1(In1), abc2alphabeta/2(b)
  Gain4/1 -> rms2/1(In1), abc2alphabeta/3(c)
  Gain5/1 -> rms3/1(In1), "abc2alphabeta "/1(a)
  Gain6/1 -> rms4/1(In1), "abc2alphabeta "/2(b)
  Gain7/1 -> rms5/1(In1), "abc2alphabeta "/3(c)
  Gain8/1 -> [pwr_act_grid]
  Gain9/1 -> [pwr_react_grid]
  [ugd_abc_pu] -> Demux2/1
  [igd_abc_pu] -> Demux3/1
  Bus Creator/1 -> [u_grid_pu_rms]
  rms4/1(Out1) -> Bus Creator1/2  "ib_grid_pu_rms"
  rms3/1(Out1) -> Bus Creator1/1  "ia_grid_pu_rms"
  rms5/1(Out1) -> Bus Creator1/3  "ic_grid_pu_rms"
  Bus Creator1/1 -> [i_grid_pu_rms]
  [cos_phi_avg] -> Terminator/1

== system afe_inv_psm_with_hf_models/afe_abc_inv_psm_mod1/AFE_control/afe_control/interesting scopes ==
  current_sequences_mod1 : Scope  NumInputPorts=4
      settings: ActiveDisplayYMinimum=-0.97178065031766891  ActiveDisplayYMaximum=1.9392475411295891  DataLoggingVariableName=ScopeData2
  i_grid_seq_ref : Scope
      settings: ActiveDisplayYMinimum=-1.1499999999999995  ActiveDisplayYMaximum=0.34999999999999981
  voltage_sequences_mod1 : Scope  NumInputPorts=4
      settings: ActiveDisplayYMinimum=-1.2405151816982258  ActiveDisplayYMaximum=1.2605257614333911
  wires:
  [v_grid_neg_eta_avg] -> voltage_sequences_mod1/4  "u_grid_neg_eta"
  [i_grid_neg_xi_avg] -> current_sequences_mod1/3  "i_grid_neg_xi"
  [v_grid_pos_eta_avg] -> voltage_sequences_mod1/2  "u_grid_pos_eta"
  [v_grid_neg_xi_avg] -> voltage_sequences_mod1/3  "u_grid_neg_xi"
  [i_grid_pos_xi_avg] -> current_sequences_mod1/1  "i_grid_pos_xi"
  [i_grid_neg_eta_avg] -> current_sequences_mod1/4  "i_grid_neg_eta"
  [v_grid_pos_xi_avg] -> voltage_sequences_mod1/1  "u_grid_pos_xi"
  [i_grid_pos_eta_avg] -> current_sequences_mod1/2  "i_grid_pos_eta"
  [i_grid_seq_ref] -> i_grid_seq_ref/1  "i_grid_seq_ref"

== system afe_inv_psm_with_hf_models/afe_abc_inv_psm_mod1/AFE_control/afe_control/is afe quantizzation and one step delay ==
  is_abc_pu : Inport
  Demux : Demux  Outputs=3
  Mux : Mux  Inputs=3
  is afe quantizzation and one step delay : Subsystem
  isd_abc_pu : Outport
  wires:
  is afe quantizzation and one step delay/2(isd_v_pu) -> Mux/2
  is_abc_pu/1 -> Demux/1
  is afe quantizzation and one step delay/3(isd_w_pu) -> Mux/3
  is afe quantizzation and one step delay/1(isd_u_pu) -> Mux/1
  Demux/1 -> is afe quantizzation and one step delay/1(is_u_pu)
  Mux/1 -> isd_abc_pu/1
  Demux/3 -> is afe quantizzation and one step delay/3(is_w_pu)
  Demux/2 -> is afe quantizzation and one step delay/2(is_v_pu)

== system afe_inv_psm_with_hf_models/afe_abc_inv_psm_mod1/AFE_control/afe_control/islanding_mode_detector ==
  gamma : Inport
  alpha : Inport  Port=2
  beta : Inport  Port=3
  Gain : Gain  Gain=7
  MATLAB Function : MATLAB Function  TreatAsAtomicUnit=on
  Terminator : Terminator
  Terminator1 : Terminator
  bounder : MATLAB Function  TreatAsAtomicUnit=on
  moving_avarage_1 : Subsystem
  moving_avarage_2 : Subsystem
  seventh_ugrid_component : Scope  NumInputPorts=2
      settings: ActiveDisplayYMinimum=-0.0034745064787606167  ActiveDisplayYMaximum=0.0074022094547510631  DataLoggingVariableName=ScopeData10
  tag scope: u_7th_eta_avg=scoped, u_7th_xi_avg=scoped
  wires:
  gamma/1 -> Gain/1  "gamma_grid"
  MATLAB Function/1(xi) -> moving_avarage_1/1(u)
  bounder/1(y) -> MATLAB Function/3(gamma)
  Gain/1 -> bounder/1(u)
  alpha/1 -> MATLAB Function/1(alpha)  "u_grid_alpha"
  beta/1 -> MATLAB Function/2(beta)  "u_grid_beta"
  MATLAB Function/2(eta) -> moving_avarage_2/1(u)
  moving_avarage_1/1(y) -> [u_7th_xi_avg], seventh_ugrid_component/1  "u_7th_xi"
  moving_avarage_2/1(y) -> [u_7th_eta_avg], seventh_ugrid_component/2  "u_7th_eta"
  [u_7th_xi_avg] -> Terminator/1
  [u_7th_eta_avg] -> Terminator1/1

== system afe_inv_psm_with_hf_models/afe_abc_inv_psm_mod1/AFE_control/afe_control/phase_compensation_1 ==
  local_time : Inport
  master_time : Inport  Port=2
  Zero-Order Hold : ZeroOrderHold  SampleTime=-1
  Zero-Order Hold1 : ZeroOrderHold  SampleTime=-1
  alignment_eval_afe1 : Subsystem
  y : Outport
  wires:
  local_time/1 -> Zero-Order Hold/1
  master_time/1 -> Zero-Order Hold1/1
  alignment_eval_afe1/1(dp) -> y/1
  Zero-Order Hold/1 -> alignment_eval_afe1/1(local_time)
  Zero-Order Hold1/1 -> alignment_eval_afe1/2(master_time)

== system afe_inv_psm_with_hf_models/afe_abc_inv_psm_mod1/AFE_control/afe_control/space_vector ==
  uab_out : Inport
  Bus Creator : BusCreator  Inputs=3
  Bus Selector : BusSelector  OutputSignals=da,db,dc
  Bus Selector1 : BusSelector  OutputSignals=ualpha_afe,ubeta_afe,ugamma_afe
  C Caller : CCaller  FunctionName=sv_pwm_cm_process_simulink  PortSpecificationStruct="%)30     .    B H   8    (     @         %    \"     8    !     0         %  0 \"0    $    _    07)G3F%M90  4&]R=$YA;64 4V-O<&4     26YD97@     5'EP90      4VEZ90      27-';&]B86P   X    P    !@    @    $          4    (     0    ,    !         !   P!O=70 #@   #     &    \"     0         !0    @    !     P    $         $  # &]U=  .    .     8    (    !          %    \"     $    &     0         0   ...(+3252 chars)"
  Constant : Constant  Value=glb_time.ts_afe
  Constant1 : Constant
  Data Type Conversion1 : DataTypeConversion  OutDataTypeStr=double  SaturateOnIntegerOverflow=off  RndMeth=Floor
  Data Type Conversion{4,15..16,18} (4 alike) : DataTypeConversion  OutDataTypeStr=single  SaturateOnIntegerOverflow=off  RndMeth=Floor
  Data Type Conversion17 : DataTypeConversion  OutDataTypeStr=uint32  SaturateOnIntegerOverflow=off  RndMeth=Floor
  Data Type Conversion2 : DataTypeConversion  OutDataTypeStr=double  SaturateOnIntegerOverflow=off  RndMeth=Floor
  Data Type Conversion3 : DataTypeConversion  OutDataTypeStr=double  SaturateOnIntegerOverflow=off  RndMeth=Floor
  Gain1 : Gain  Gain=sqrt(3)/2
  Gain2 : Gain  Gain=sqrt(3)/2
  Gain3 : Gain  Gain=u_cm_comp_mod1
  duvw : Outport
  wires:
  Data Type Conversion15/1 -> C Caller/2
  Bus Selector/2 -> Data Type Conversion2/1  "<db>"
  Data Type Conversion18/1 -> C Caller/1
  C Caller/1 -> Bus Selector/1
  Bus Creator/1 -> duvw/1
  Data Type Conversion1/1 -> Bus Creator/1  "du(k)"
  Bus Selector1/2 -> Gain2/1  "<ubeta_afe>"
  Bus Selector/3 -> Data Type Conversion3/1  "<dc>"
  Bus Selector1/1 -> Gain1/1  "<ualpha_afe>"
  Data Type Conversion2/1 -> Bus Creator/2  "dv(k)"
  Gain2/1 -> Data Type Conversion15/1
  Bus Selector/1 -> Data Type Conversion1/1  "<da>"
  Gain1/1 -> Data Type Conversion18/1
  Data Type Conversion3/1 -> Bus Creator/3  "dw(k)"
  Constant/1 -> Data Type Conversion16/1
  uab_out/1 -> Bus Selector1/1
  Constant1/1 -> Data Type Conversion17/1
  Data Type Conversion16/1 -> C Caller/4
  Data Type Conversion17/1 -> C Caller/5
  Bus Selector1/3 -> Gain3/1  "<ugamma_afe>"
  Gain3/1 -> Data Type Conversion4/1
  Data Type Conversion4/1 -> C Caller/3

== system afe_inv_psm_with_hf_models/afe_abc_inv_psm_mod1/AFE_control/afe_control/udc_acquisition ==
  udc_pu : Inport
  Quantizer : Quantizer  QuantizationInterval=adc_quantization
  Unit Delay : UnitDelay  SampleTime=-1
  Zero-Order Hold : ZeroOrderHold  SampleTime=-1
  udcd_pu : Outport
  wires:
  Quantizer/1 -> Unit Delay/1
  udc_pu/1 -> Zero-Order Hold/1
  Unit Delay/1 -> udcd_pu/1
  Zero-Order Hold/1 -> Quantizer/1

== system afe_inv_psm_with_hf_models/afe_abc_inv_psm_mod1/AFE_control/afe_control/udc_ctrl ==
  udc_pu : Inport
  1/Ti : Gain  Gain=afe_ctrl.kp_udc_ctrl  SaturateOnIntegerOverflow=on  OutDataTypeStr=Inherit: Same as input  ParamDataTypeStr=Inherit: Same as input
  Constant : Constant  Value=0
  Gain : Gain  Gain=-1
  Saturation : Saturate  UpperLimit=afe_ctrl.ixi_pos_ref_lim  LowerLimit=-afe_ctrl.ixi_pos_ref_lim
  Sum1 : Sum  Inputs=+++  SaturateOnIntegerOverflow=on
  Sum2 : Sum  Inputs=-+  SaturateOnIntegerOverflow=on
  Sum3 : Sum  Inputs=-+  SaturateOnIntegerOverflow=on
  Switch : Switch  Criteria=u2 > Threshold  SaturateOnIntegerOverflow=off  InputSameDT=off
  To Workspace1 : ToWorkspace  VariableName=udc_pu_sim_mod1  SampleTime=-1
      settings: MaxDataPoints=glb_time.Ns_afe
  To Workspace3 : ToWorkspace  VariableName=udc_pu_ref_sim_mod1  SampleTime=-1
      settings: MaxDataPoints=glb_time.Ns_afe
  Unit Delay4 : UnitDelay  SampleTime=-1
  discrete-time-low-pass-filter1 : discrete_time_low_pass_filter/discrete-time-low-pass-filter  tau=20e-3  ts=glb_time.ts_afe
  kp : Gain  Gain=afe_ctrl.ki_udc_ctrl*glb_time.ts_afe  SaturateOnIntegerOverflow=on  OutDataTypeStr=Inherit: Same as input  ParamDataTypeStr=Inherit: Same as input
  udc_norm_ref : Step  Time=1e-3  FinalValue=afe_ctrl.udc_norm_ref
  udc_tracking : Scope  NumInputPorts=3
      settings: ActiveDisplayYMinimum=-2.0004150390624997  ActiveDisplayYMaximum=1.5037353515624998  DataLoggingVariableName=ScopeData8
  i_xi_ref : Outport
  wires:
  1/Ti/1 -> Sum1/1, Sum3/1
  kp/1 -> Sum1/2
  Sum3/1 -> Unit Delay4/1
  Unit Delay4/1 -> Sum1/3
  udc_norm_ref/1 -> discrete-time-low-pass-filter1/1
  udc_pu/1 -> Sum2/1, To Workspace1/1, udc_tracking/2  "udc_pu"
  Sum2/1 -> kp/1, 1/Ti/1
  Sum1/1 -> Saturation/1
  [pwr_lim_enable] -> Switch/2
  Saturation/1 -> Switch/3
  Switch/1 -> Sum3/2, Gain/1
  Constant/1 -> Switch/1
  Gain/1 -> udc_tracking/3, i_xi_ref/1  "i_xi_ref"
  discrete-time-low-pass-filter1/1 -> To Workspace3/1, udc_tracking/1, Sum2/2  "udc_pu_ref"

== system afe_inv_psm_with_hf_models/afe_abc_inv_psm_mod1/AFE_control/afe_control/ug afe quantizzation and one step delay ==
  ug_abc_pu : Inport
  Demux : Demux  Outputs=3
  Mux : Mux  Inputs=3
  ug afe quantizzation and one step delay : Subsystem
  ugd_abc_pu : Outport
  wires:
  ug afe quantizzation and one step delay/2(ugd_v_pu) -> Mux/2
  Demux/2 -> ug afe quantizzation and one step delay/2(ug_v_pu)
  Demux/3 -> ug afe quantizzation and one step delay/3(ug_w_pu)
  ug afe quantizzation and one step delay/1(ugd_u_pu) -> Mux/1
  Demux/1 -> ug afe quantizzation and one step delay/1(ug_u_pu)
  ug_abc_pu/1 -> Demux/1
  ug afe quantizzation and one step delay/3(ugd_w_pu) -> Mux/3
  Mux/1 -> ugd_abc_pu/1

== system afe_inv_psm_with_hf_models/afe_abc_inv_psm_mod1/INV_control/inverter_control/Speed control ==
  rotor speed : Inport
  rotor speed ref : Inport  Port=2
  1/Ti : Gain  Gain=psm_ctrl.kp_w  SaturateOnIntegerOverflow=on  OutDataTypeStr=Inherit: Same as input  ParamDataTypeStr=Inherit: Same as input
  Saturation : Saturate  UpperLimit=psm_ctrl.iq_lim  LowerLimit=-psm_ctrl.iq_lim
  Sum1 : Sum  Inputs=+++  SaturateOnIntegerOverflow=on
  Sum2 : Sum  Inputs=-+  SaturateOnIntegerOverflow=on
  Sum3 : Sum  Inputs=-+  SaturateOnIntegerOverflow=on
  Unit Delay4 : UnitDelay  SampleTime=-1
  kp : Gain  Gain=psm_ctrl.ki_w*glb_time.ts_inv  SaturateOnIntegerOverflow=on  OutDataTypeStr=Inherit: Same as input  ParamDataTypeStr=Inherit: Same as input
  torque_ref : Outport
  wires:
  1/Ti/1 -> Sum1/1, Sum3/1
  kp/1 -> Sum1/2
  Sum3/1 -> Unit Delay4/1
  Unit Delay4/1 -> Sum1/3
  rotor speed ref/1 -> Sum2/2
  rotor speed/1 -> Sum2/1
  Sum2/1 -> kp/1, 1/Ti/1
  Sum1/1 -> Saturation/1
  Saturation/1 -> Sum3/2, torque_ref/1

== system afe_inv_psm_with_hf_models/afe_abc_inv_psm_mod1/INV_control/inverter_control/current_ctrl ==
  torque_ref : Inport
  Bus Creator1 : BusCreator  Inputs=2
  bemf_observer : Subsystem
  current_ctrl : Subsystem
  current_transformation : Subsystem
  uab : Outport  VectorParamsAs1DForOutWhenUnconnected=off
  wires:
  [ubeta_pu_mod1] -> Bus Creator1/2  "ub"
  [ualpha_pu_mod1] -> Bus Creator1/1  "ua"
  Bus Creator1/1 -> uab/1
  torque_ref/1 -> current_ctrl/1(iq_ref)  "torque_ref"
  [ibeta_pu_mod1] -> bemf_observer/2(ibeta_pu)
  [ialpha_pu_mod1] -> bemf_observer/1(ialpha_pu)
  [ualpha_pu_mod1] -> bemf_observer/3(ualpha_pu)
  [ubeta_pu_mod1] -> bemf_observer/4(ubeta_pu)
  [udcd_pu_inv_mod1] -> current_ctrl/2(udc_pu), bemf_observer/5(udc_pu)

== system afe_inv_psm_with_hf_models/afe_abc_inv_psm_mod1/INV_control/inverter_control/encoder-sensorless-switch ==
  Constant : Constant  Value=psm_ctrl.omega_th
  MATLAB Function : MATLAB Function  TreatAsAtomicUnit=on
  Variant Source1 : VariantSource  VariantControls={use_psm_encoder == 1, use_psm_encoder == 0}
  Variant Source2 : VariantSource  VariantControls={use_psm_encoder == 1, use_psm_encoder == 0}
  double_integrator_observer : Subsystem
  omega_pu_psm/hat1 : Scope  NumInputPorts=2
      settings: ActiveDisplayYMinimum=-2.3213334849146574  ActiveDisplayYMaximum=1.1003523731757916  DataLoggingVariableName=ScopeData13
  phase_elec_psm/hat : Scope  NumInputPorts=2
      settings: ActiveDisplayYMinimum=-3.926950967479629  ActiveDisplayYMaximum=3.92663217141873  DataLoggingVariableName=ScopeData12
  tag scope: motor_phase_ctrl_mod1=scoped, motor_speed_pu_ctrl_mod1=scoped
  wires:
  Variant Source1/1 -> [motor_speed_pu_ctrl_mod1]
  Variant Source2/1 -> [motor_phase_ctrl_mod1]
  [phase_hat_mod1] -> phase_elec_psm/hat/1  "theta_hat_mod1"
  [omega_hat_pu_mod1] -> omega_pu_psm/hat1/1  "omega_hat_pu_mod1"
  [phased_psm] -> double_integrator_observer/1(phase_psm)
  MATLAB Function/1(omega_ctrl) -> Variant Source1/2
  MATLAB Function/2(phase_ctrl) -> Variant Source2/2
  double_integrator_observer/1(phase_psm_hat) -> phase_elec_psm/hat/2, Variant Source2/1, MATLAB Function/1(phase_psm)  "phase_psm_hat"
  double_integrator_observer/2(omega_pu_psm_hat) -> Variant Source1/1, omega_pu_psm/hat1/2, MATLAB Function/2(omega_obs)  "omega_pu_psm_hat"
  [phase_hat_mod1] -> MATLAB Function/3(phase_obs)  "theta_hat_mod1"
  [omega_hat_pu_mod1] -> MATLAB Function/4(omega_psm)  "omega_hat_pu_mod1"
  Constant/1 -> MATLAB Function/5(omega_th)
